simulink model "ACMFDS_Stateflow"  (R2024a)
settings: Solver=VariableStepAuto  StartTime=0.0  StopTime=inf  RelTol=1e-3
settings Model: Creator=VARUN  LastModifiedBy=VARUN

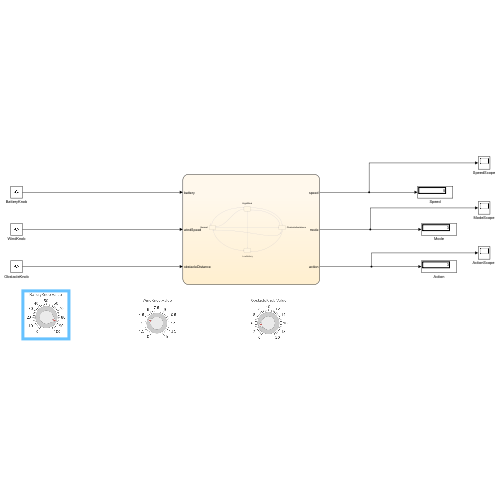
[thumbnail: Simulink's stored preview of the top-level diagram]
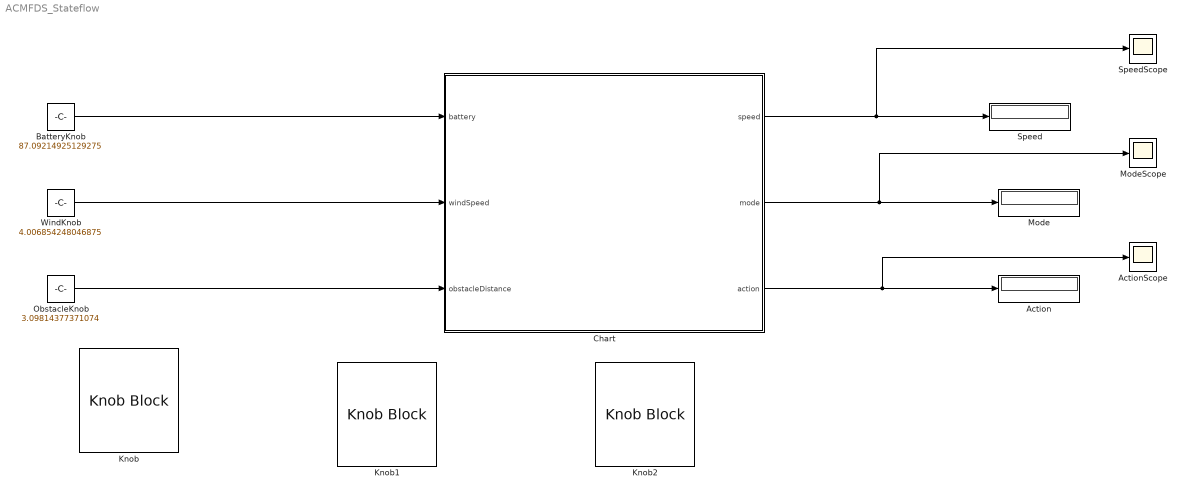
== system ACMFDS_Stateflow ==
  Action : Display
  "ActionScope " : Scope
  BatteryKnob : Constant  Value=87.09214925129275
  Chart : Stateflow chart  TreatAsAtomicUnit=on
  Knob : KnobBlock
  Knob1 : KnobBlock  ScaleMax=15
  Knob2 : KnobBlock  ScaleMax=20
  Mode : Display
  ModeScope : Scope
  ObstacleKnob : Constant  Value=3.09814377371074
  Speed : Display
  SpeedScope : Scope
  WindKnob : Constant  Value=4.006854248046875
  wires:
  Chart/1(speed) -> SpeedScope/1, Speed/1
  Chart/3(action) -> "ActionScope "/1, Action/1
  ObstacleKnob/1 -> Chart/3(obstacleDistance)
  WindKnob/1 -> Chart/2(windSpeed)
  BatteryKnob/1 -> Chart/1(battery)
  Chart/2(mode) -> ModeScope/1, Mode/1

== stateflow chart ACMFDS_Stateflow/Chart ==
  note: HighWind
  state entry_1
    speed = 7;
    mode = 2;
    action = 2;
  state entry_
    speed = 10;
    mode = 1;
    action = 1;
  state entry_2
    speed = 5;
    mode = 3;
    action = 3;
  note: Normal
  note: ObstacleAvoidance
  state entry_3
    speed = 4;
    mode = 4;
    action = 4;
  note: LowBattery
  entry_ -> entry_1 [order 1] : [windSpeed >= 10 && obstacleDistance > 5 && battery > 20]
  entry_1 -> entry_2 [order 2] : [obstacleDistance <= 5 && battery > 20]
  entry_1 -> entry_ [order 1] : [windSpeed < 10 && obstacleDistance > 5 && battery > 20]
  entry_2 -> entry_1 [order 2] : [obstacleDistance > 5 && windSpeed >= 10 && battery > 20]
  entry_3 -> entry_1 [order 1] : [obstacleDistance >5 && windSpeed <10 &&battery >20]
  entry_1 -> entry_3 [order 3] : [battery <= 20]
  (default) -> entry_
  entry_ -> entry_2 [order 2] : [obstacleDistance <= 5 && battery > 20]
  entry_3 -> entry_ [order 3] : [battery >20 && windSpeed <10 && obstacleDistance>5]
  entry_2 -> entry_ [order 1] : [obstacleDistance > 5 && windSpeed < 10 && battery > 20]
  entry_ -> entry_3 [order 3] : [battery <= 20]
  entry_2 -> entry_3 [order 3] : [battery <= 20]
  entry_3 -> entry_2 [order 2] : [battery >20 && obstacleDistance <=5]
  data: speed output; mode output; action output; battery input; windSpeed input; obstacleDistance input
